simulink model "thermobox_Open_Loop"  (R2026a)
settings: Solver=VariableStepAuto  StopTime=2000
settings Model: Creator=dvyse  LastModifiedBy=dvyse
settings OptimizationCC: BufferReuse=off

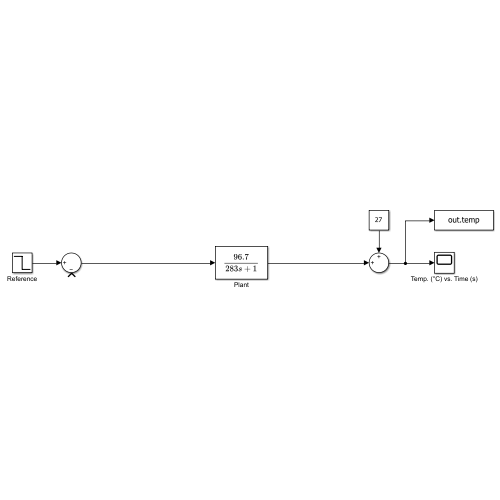
[thumbnail: Simulink's stored preview of the top-level diagram]
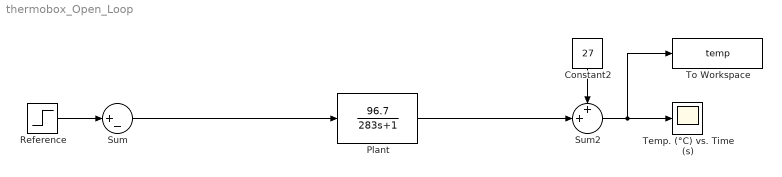
== system thermobox_Open_Loop ==
  Constant2 : Constant  Value=27
  Plant : TransferFcn  Numerator=[96.7]  Denominator=[283 1]
  Reference : Step  Time=0  InitialValue=27  SampleTime=0
  Sum : Sum  Inputs=|+-
  Sum2 : Sum  Inputs=++|
  Temp. (°C) vs. Time (s) : Scope
      settings: ActiveDisplayYMinimum=-14.097172899886615  ActiveDisplayYMaximum=155.84106575121393
  To Workspace : ToWorkspace  VariableName=temp  SaveFormat=Timeseries  SampleTime=-1
  wires:
  Plant/1 -> Sum2/2
  Reference/1 -> Sum/1
  Sum/1 -> Plant/1
  Sum2/1 -> To Workspace/1, Temp. (°C) vs. Time (s)/1
  Constant2/1 -> Sum2/1
